simulink model "QD2_Sim_Dual"  (R2022a)
settings: Solver=FixedStepDiscrete  StartTime=0.0  StopTime=400  FixedStep=0.002  RelTol=1e-3
PreLoadFcn:
  | % QD2_Sim_Dual: agrega lib/ y sim/ al path antes de cargar (enlaces a QD2_Mission_Lib)
  | qd2_c = {pwd};
  | qd2_w = which('QD2_Sim_Dual');
  | if ~isempty(qd2_w), qd2_c{end+1} = fileparts(qd2_w); end
  | for qd2_i = 1:numel(qd2_c)
  |     qd2_d = qd2_c{qd2_i};
  |     for qd2_k = 1:4
  |         if exist(fullfile(qd2_d, 'lib', 'QD2_Mission_Lib.slx'), 'file')
  |             addpath(fullfile(qd2_d, 'lib'));
  |             addpath(fullfile(qd2_d, 'sim'));
  |             break;
  |         end
  |         qd2_d = fileparts(qd2_d);
  |     end
  | end
  | clear qd2_c qd2_w qd2_i qd2_d qd2_k
PostLoadFcn:
  | % QD2_Sim_Dual: rutas de lib/ (funciones qd2_* y QD2_Mission_Lib) y sim/
  | qd2_d = fileparts(get_param(bdroot, 'FileName'));
  | for qd2_k = 1:4
  |     if exist(fullfile(qd2_d, 'lib', 'qd2_params.m'), 'file'), break; end
  |     qd2_d = fileparts(qd2_d);
  | end
  | addpath(fullfile(qd2_d, 'lib'));
  | addpath(fullfile(qd2_d, 'sim'));
  | clear qd2_d qd2_k
InitFcn:
  | % QD2_Sim_Dual: rutas de lib/ (funciones qd2_* y QD2_Mission_Lib) y sim/
  | qd2_d = fileparts(get_param(bdroot, 'FileName'));
  | for qd2_k = 1:4
  |     if exist(fullfile(qd2_d, 'lib', 'qd2_params.m'), 'file'), break; end
  |     qd2_d = fileparts(qd2_d);
  | end
  | addpath(fullfile(qd2_d, 'lib'));
  | addpath(fullfile(qd2_d, 'sim'));
  | clear qd2_d qd2_k
  | % Parámetros (config/estacion.json es la única fuente de verdad)
  | QD2P = qd2_params_from_config();
  | QD2_SIM = qd2_sim_parametros();
  | % La versión la fija el bloque constante VERSION de la raíz
  | QD2_VERSION = str2double(get_param([bdroot '/' sprintf('VERSION\n(1 = PID, 2 = MPC)')], 'Value'));
libraries: simulink x1
(part 1 of 2)
settings Model: ExtModeTrigDuration=10000  Creator=ezequ  LastModifiedBy=ezequ
settings SolverCC: AlgebraicLoopSolver=TrustRegion  PositivePriorityOrder=on
settings DataIOCC: SaveFormat=Array  SaveOutput=off  SignalLogging=off  SaveTime=off
settings OptimizationCC: LifeSpan=inf
settings DebuggingCC: AlgebraicLoopMsg=error  UnconnectedInputMsg=warning  UnconnectedOutputMsg=warning  UnconnectedLineMsg=warning  ArithmeticOperatorsInVariantConditions=warning
settings SFSimCC: SimUseLocalCustomCode=off  CustomCodeUndefinedFunction=UseInterfaceOnly
settings RTWCC: Description=QUARC Win64 Target  SystemTargetFile=quarc_win64.tlc  TemplateMakefile=quarc_default_tmf  RTWUseLocalCustomCode=off
settings CodeAppCC: StateflowObjectComments=on
settings STFCustomTargetCC: TargetPreCompLibLocation=C:\PROGRA~3\QUARC\lib\2016a\win64\release  TargetLangStandard=C99 (ISO)  ConcurrentExecutionCompliant=on  SystemTargetFile=quarc_win64.tlc
settings GRTTargetCC: TargetPreCompLibLocation=C:\PROGRA~3\QUARC\lib\2016a\win64\release  ParMdlRefBuildCompliant=off  CompOptLevelCompliant=off  CombineOutputUpdateFcns=off  MatFileLogging=off  CPPClassGenCompliant=off  GRTInterface=on  UseToolchainInfoCompliant=off  ExtMode=on  ExtModeMexFile=quarc_comm
settings ConfigComp: CovMetricSettings=dswe  CovBoundaryAbsTol=1.0e-5

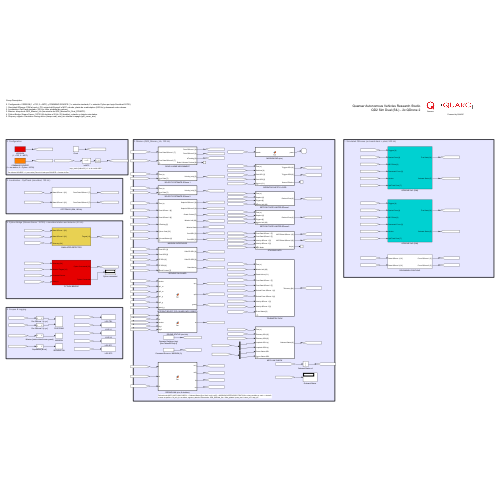
[thumbnail: Simulink's stored preview of the top-level diagram]
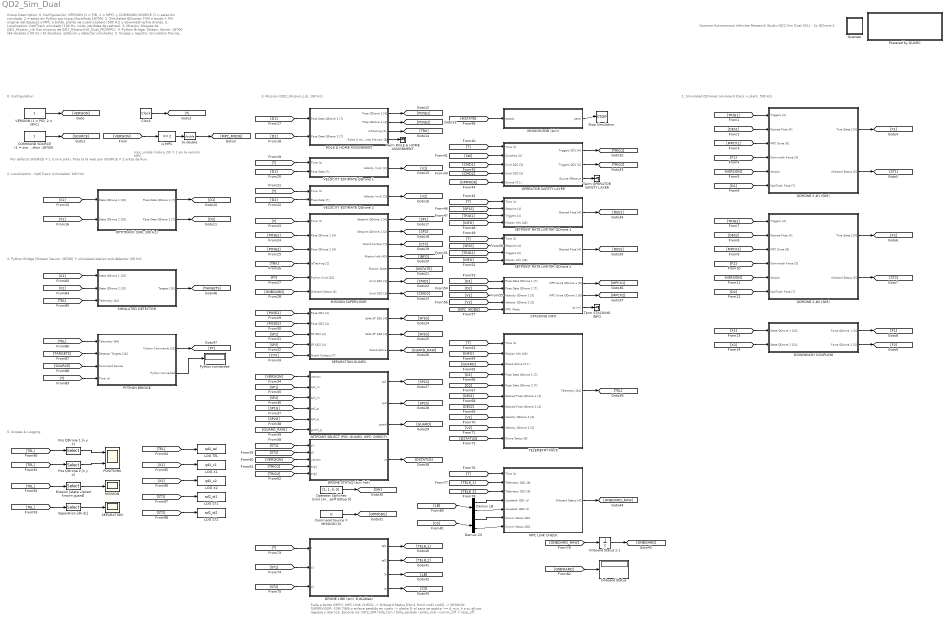
== system QD2_Sim_Dual ==
  note: Group Description:
      |
      | 0. Configuración: VERSION (1 = PID, 2 = MPC) y COMMAND SOURCE (1 = estación simulada, 2 = estación Python por tcpip://localhost:18700).
      | 1. Simulated QDrones: FSM a bordo + PIV original del Equipo2 o MPC a bordo, planta de cuadricóptero (500 Hz) y downwash entre drones.
      | 2. Localization: OptiTrack simulado (100 Hz, ruido, pérdidas de rastreo).
      | 3. Mission: bloques de QD2_Mission_Lib (los mismos de QD2_MissionCtrl_Dual_PID/MPC).
      | 4. Python Bridge: Stream Server :18700 (64 doubles a 50 Hz / 32 doubles), estación y detector simulados.
      | 5. Scopes y registro. Simulation Pacing activo (tiempo real); sim() sin interfaz lo apaga (qd2_correr_sim).
  note: Quanser Autonomous Vehicles Research Studio
      | QD2 Sim Dual (SIL) - 2x QDrone 2
  note: 0. Configuration
  note: mpc_mode (índice 23) = 1 en la versión MPC
  note: Por defecto SOURCE = 1 (corre sola). Para la UI web pon SOURCE = 2 antes de Run.
  note: 1. Simulated QDrones (on-board stack + plant, 500 Hz)
  note: 2. Localization - OptiTrack (simulated, 100 Hz)
  note: 3. Mission (QD2_Mission_Lib, 100 Hz)
  note: Falla a bordo (MPC): MPC LINK CHECK -> Onboard Status [fsm1 fsm2 cod1 cod2] -> MISSION SUPERVISOR. FSM 7/8/9 o enlace perdido en vuelo -> alerta 9:
      | el sano se aparta >= d_min_h a su altura, regresa y aterriza. Escenarios: QD2_SIM.falla_fsm / falla_apilado / proto_mal / comm_off + resp_off.
  note: 4. Python Bridge (Stream Server :18700) + simulated station and detector (50 Hz)
  note: 5. Scopes & Logging
  "COMMAND SOURCE (1 = sim station, 2 = Python :18700)" : Constant
  Clock : DigitalClock  SampleTime=0.01
  Command Source = MISSION (0) : Constant  Value=0  SampleTime=0.01
  DOWNWASH COUPLING : Subsystem
  "DRONE LINK (sim, 8 doubles)" : MATLAB Function  TreatAsAtomicUnit=on
  DRONE STATUS (sim link) : MATLAB Function  TreatAsAtomicUnit=on
  Demux CS : Demux  Outputs=2
  Demux LB : Demux  Outputs=2
  LOG ST1 : ToWorkspace  VariableName=qd2_st1  SampleTime=0.02
  LOG ST2 : ToWorkspace  VariableName=qd2_st2  SampleTime=0.02
  LOG TEL : ToWorkspace  VariableName=qd2_tel  SampleTime=0.02
  LOG X1 : ToWorkspace  VariableName=qd2_x1  SampleTime=0.02
  LOG X2 : ToWorkspace  VariableName=qd2_x2  SampleTime=0.02
  MISSION : Scope
  MISSION END (sim) : MATLAB Function  TreatAsAtomicUnit=on
  MISSION SUPERVISOR : Subsystem  TreatAsAtomicUnit=on  SystemSampleTime=Ts  mask(QD2 Mission Lib){P=QD2P, version=QD2_VERSION, Ts=0.01}
      mask prompts: P "Parámetros de misión (struct de qd2_params_from_config):"; version "Versión (1 = PID, 2 = MPC):"; Ts "Paso de muestreo (s):"
      mask help: FSM de misión (qd2_mission_step, ARQUITECTURA §3.3). Commands = [arm takeoff estop] por dron: el OPERATOR SAFETY LAYER los combina con los switches del operador. Guard Context = [explorer_id ctx_guard(6)]. Onboard Status [4] = [fsm1 fsm2 cod1 cod2] del MPC LINK CHECK (versión MPC; en PID constante 0 = desconocido; cod 1 = protocolo MPC incorrecto, 2 = enlace perdido): un dron en vuelo con FSM a bordo 7/8/9 o sin enlace (o protocolo incorrecto) -> alerta 9 (10), el sano se aparta >= d_min_h a su altura, regresa y aterriza; DONE. En LANDING, R no baja hasta que E está a >= d_min_h en horizontal. Mission Info [40] = campos de telemetría para el TELEMETRY PACK (ver codigo_supervisor en construir_modelos.m).
  MPC LINK CHECK : Subsystem  TreatAsAtomicUnit=on  SystemSampleTime=Ts  mask(QD2 Mission Lib){P=QD2P, version=QD2_VERSION, Ts=0.01}
      mask prompts: P "Parámetros de misión (struct de qd2_params_from_config):"; version "Versión (1 = PID, 2 = MPC):"; Ts "Paso de muestreo (s):"
      mask help: Versión MPC (qd2_enlace_mpc): valida la respuesta de 8 doubles de cada dron (§3.2): válida si y(8) = 2 (etiqueta protocolo MPC v1) y la FSM y(2) es un entero 1..9. Si el dron está conectado (loopback < 0.5 s y sin pérdida de enlace) y responde mal más de 0.5 s seguidos -> protocolo incorrecto (cod 1, alerta 10, dron no disponible). Sin conexión después de haber estado conectado -> enlace perdido (cod 2; la FSM retenida no se usa: fsm = 0). Onboard Status = [fsm1 fsm2 cod1 cod2] (fsm 0 = desconocida) -> MISSION SUPERVISOR. Con version = 1 (PID, el dron solo devuelve el eco) la salida es 0.
  Mission [state visited known guard] : Selector  InputPortWidth=64  IndexOptions=Index vector (dialog)  Indices=[2 10 9 11]  OutputSizes=1
  OPERATOR SAFETY LAYER : Subsystem  TreatAsAtomicUnit=on  SystemSampleTime=Ts  mask(QD2 Mission Lib){Ts=0.01}
      mask prompts: Ts "Paso de muestreo (s):"
      mask help: Versión SIMPLE (la usa QD2_Sim_Dual; interfaz de 5/3 puertos sin cambios). Los modelos de tierra usan OPERATOR SAFETY LAYER DUAL. En modo MISIÓN (Command Source = 0) arm_i = switch AND misión, takeoff_i = switch AND misión (solo tras >= 1 s armado), estop_i = switch OR misión. En modo MANUAL Equipo2 (1) el dron 1 recibe los switches (takeoff también >= 1 s después de armar) y el dron 2 solo el E-stop. El modo solo cambia con los dos drones desarmados Y los switches Arm y Takeoff abajo (nunca se dispara solo).
  "OPTITRACK (SIM, 100 Hz)" : Subsystem
  Onboard Status : Display
  Onboard Status z-1 : UnitDelay  InitialCondition=[0; 0; 0; 0]  SampleTime=0.01  HasFrameUpgradeWarning=on
  Operator Switches (sim) [Arm Takeoff EStop 0] : Constant  Value=[1; 1; 0; 0]  SampleTime=0.01
  POSITIONS : Scope  NumInputPorts=2
  PYTHON BRIDGE : Subsystem
  Pos QDrone 1 [x y z] : Selector  InputPortWidth=64  IndexOptions=Index vector (dialog)  Indices=[17 18 19]  OutputSizes=1
  Pos QDrone 2 [x y z] : Selector  InputPortWidth=64  IndexOptions=Index vector (dialog)  Indices=[35 36 37]  OutputSizes=1
  Powered by QUARC : Subsystem  mask(Powered by QUARC){}
      mask help: Double-clicking the block will open the QUARC web site.
      settings: OpenFcn=web('https://www.quanser.com/products/quarc-real-time-control-software/', '-browser');
      mask Help: web(qc_get_block_help_path(gcb));
      mask Display: image(imread(fullfile(qc_root, 'blocks', 'quarc_logo.png')));
  Python connected : Display
  QDRONE 2 #1 (SIM) : Subsystem
  QDRONE 2 #2 (SIM) : Subsystem
  Quanser : Subsystem  mask(Powered by Quanser){}
      mask help: Double-clicking the block will open the Quanser web site.
      settings: OpenFcn=web('http://www.quanser.com', '-browser');
      mask Help: web(qc_get_block_help_path(gcb));
      mask Display: image(imread(fullfile(qc_root, 'blocks', 'quanser_logo.jpg')));
  ROLE & HOME ASSIGNMENT : Subsystem  TreatAsAtomicUnit=on  SystemSampleTime=Ts  mask(QD2 Mission Lib){P=QD2P, version=QD2_VERSION, Ts=0.01}
      mask prompts: P "Parámetros de misión (struct de qd2_params_from_config):"; version "Versión (1 = PID, 2 = MPC):"; Ts "Paso de muestreo (s):"
      mask help: Separa [x y z yaw] e isTracking de cada dron (Corrected Pose Data [7] = [x y z roll pitch yaw isTracking]) y muestra en vivo la asignación de roles de qd2_assign_roles: [explorer_id responder_id home1(2) home2(2) d_homes start_ok]. El dron con menor x es el EXPLORADOR. El MISSION SUPERVISOR fija roles y homes al recibir START; start_ok = 0 avisa ANTES de START que los homes están demasiado cerca (START se rechazaría, alerta 1).
  SEPARATION : Scope
  SEPARATION GUARD : Subsystem  TreatAsAtomicUnit=on  SystemSampleTime=Ts  mask(QD2 Mission Lib){P=QD2P, Ts=0.01}
      mask prompts: P "Parámetros de misión (struct de qd2_params_from_config):"; Ts "Paso de muestreo (s):"
      mask help: Versión PID: nunca uno encima del otro (qd2_separation_guard). Distancia horizontal >= d_min_h entre poses, consignas y caminos rectos. Traduce dron <-> rol con explorer_id (Guard Context(1)) y reinicia su estado si los roles cambian. Después de este bloque la consigna DEBE limitarse por norma (SETPOINT RATE LIMITER).
  SETPOINT RATE LIMITER QDrone 1 : Subsystem  TreatAsAtomicUnit=on  SystemSampleTime=Ts  mask(QD2 Mission Lib){P=QD2P, dron=1, Ts=0.01}
      mask prompts: P "Parámetros de misión (struct de qd2_params_from_config):"; dron "QDrone (1 o 2):"; Ts "Paso de muestreo (s):"
      mask help: Saturation (como Saturation2 original, con z hasta P.z_max) + limitador de razón por NORMA en x,y (qd2_rate_limit(...,1)): 1/3 m/s xy, 1/6 m/s z, 30 °/s yaw. Sustituye al Rate Limiter2 por eje (que hace caminos en L y rompe la separación). Desarmado (Triggers(1) = 0) la consigna pasa sin limitar. Mientras este dron se aparta de un dron en falla a bordo (Mission Info(37 + dron) = 1) el límite xy es P.falla_rate_xy (1 m/s). Parámetro dron = 1 o 2.
  SETPOINT RATE LIMITER QDrone 2 : Subsystem  TreatAsAtomicUnit=on  SystemSampleTime=Ts  mask(QD2 Mission Lib){P=QD2P, dron=2, Ts=0.01}
      mask prompts: P "Parámetros de misión (struct de qd2_params_from_config):"; dron "QDrone (1 o 2):"; Ts "Paso de muestreo (s):"
      mask help: Saturation (como Saturation2 original, con z hasta P.z_max) + limitador de razón por NORMA en x,y (qd2_rate_limit(...,1)): 1/3 m/s xy, 1/6 m/s z, 30 °/s yaw. Sustituye al Rate Limiter2 por eje (que hace caminos en L y rompe la separación). Desarmado (Triggers(1) = 0) la consigna pasa sin limitar. Mientras este dron se aparta de un dron en falla a bordo (Mission Info(37 + dron) = 1) el límite xy es P.falla_rate_xy (1 m/s). Parámetro dron = 1 o 2.
  "SETPOINT SELECT (PID: GUARD, MPC: DIRECT)" : MATLAB Function  TreatAsAtomicUnit=on
  SIMULATED DETECTOR : Subsystem
  STACKING INFO : Subsystem  TreatAsAtomicUnit=on  SystemSampleTime=Ts  mask(QD2 Mission Lib){Ts=0.01}
      mask prompts: Ts "Paso de muestreo (s):"
      mask help: Versión MPC: índices 17-24 del mensaje de 24 doubles (§3.2) para cada dron = [x y z vx vy vz del OTRO dron, mpc_mode, 2]. El índice 24 = 2 es la etiqueta "protocolo MPC v1": el PROTOCOL CHECK a bordo solo acepta tramas con 24 = 2. Si el otro no está rastreado se mandan NaN (el MPC a bordo desactiva el feedforward de downwash).
  Separation [dh dz] : Selector  InputPortWidth=64  IndexOptions=Index vector (dialog)  Indices=[12 13]  OutputSizes=1
  Stop Simulation : Stop
  TELEMETRY PACK : Subsystem  TreatAsAtomicUnit=on  SystemSampleTime=Ts  mask(QD2 Mission Lib){version=QD2_VERSION, Ts=0.01}
      mask prompts: version "Versión (1 = PID, 2 = MPC):"; Ts "Paso de muestreo (s):"
      mask help: Arma los 64 doubles Simulink -> Python (§3.3) con qd2_telemetry_pack. Drone Status = [fsm1 fsm2 bat1 bat2 comm_issue1 comm_issue2 loopback1 loopback2 (n_peticiones alerta_operador)]; comm_ok = sin issue y loopback < 0.5 s. y(55) = alerta: la del operador (5-8) si hay, si no la del supervisor (0-4, 9 falla a bordo, 10 protocolo MPC incorrecto). y(56:60) = un objetivo por mensaje, rotando: [id clase x y estado]. y(61:63) = [roll pitch válido] del EXPLORADOR (rad), de Pose Data(4:5) del mismo dron (OptiTrack, R = Rz(yaw)Ry(pitch)Rx(roll)); 0 0 0 sin explorador, sin rastreo o con ángulos no finitos. y(64) = 0.
  Term OPERATOR SAFETY LAYER : Terminator
  Term ROLE & HOME ASSIGNMENT : Terminator
  Term STACKING INFO : Terminator
  VELOCITY ESTIMATE QDrone 1 : Subsystem  TreatAsAtomicUnit=on  SystemSampleTime=Ts  mask(QD2 Mission Lib){Ts=0.01}
      mask prompts: Ts "Paso de muestreo (s):"
      mask help: Velocidad [vx vy vz] a partir de OptiTrack: derivada entre muestras nuevas (100 Hz) + filtro de primer orden (tau = 0.04 s). Sin rastreo -> 0.
  VELOCITY ESTIMATE QDrone 2 : Subsystem  TreatAsAtomicUnit=on  SystemSampleTime=Ts  mask(QD2 Mission Lib){Ts=0.01}
      mask prompts: Ts "Paso de muestreo (s):"
      mask help: Velocidad [vx vy vz] a partir de OptiTrack: derivada entre muestras nuevas (100 Hz) + filtro de primer orden (tau = 0.04 s). Sin rastreo -> 0.
  "VERSION (1 = PID, 2 = MPC)" : Constant
  is MPC : simulink/Logic and Bit Operations/Compare To Constant  relop===  const=2  OutDataTypeStr=boolean
  to double : DataTypeConversion  OutDataTypeStr=double  SaturateOnIntegerOverflow=off  RndMeth=Floor
  wires:
  "VERSION (1 = PID, 2 = MPC)"/1 -> [VERSION]
  "COMMAND SOURCE (1 = sim station, 2 = Python :18700)"/1 -> [SOURCE]
  Clock/1 -> [T]
  is MPC/1 -> to double/1
  [VERSION] -> is MPC/1
  to double/1 -> [MPC_MODE]
  [TRIG1] -> QDRONE 2 #1 (SIM)/1(Triggers [4])
  [DES1] -> QDRONE 2 #1 (SIM)/2(Desired Pose [4])
  [MPCX1] -> QDRONE 2 #1 (SIM)/3(MPC Extra [8])
  [F1] -> QDRONE 2 #1 (SIM)/4(Downwash Force [3])
  [VERSION] -> QDRONE 2 #1 (SIM)/5(Version)
  [D1] -> QDRONE 2 #1 (SIM)/6(OptiTrack Pose [7])
  QDRONE 2 #1 (SIM)/1(True State [10]) -> [X1]
  QDRONE 2 #1 (SIM)/2(Onboard Status [5]) -> [ST1]
  [TRIG2] -> QDRONE 2 #2 (SIM)/1(Triggers [4])
  [DES2] -> QDRONE 2 #2 (SIM)/2(Desired Pose [4])
  [MPCX2] -> QDRONE 2 #2 (SIM)/3(MPC Extra [8])
  [F2] -> QDRONE 2 #2 (SIM)/4(Downwash Force [3])
  [VERSION] -> QDRONE 2 #2 (SIM)/5(Version)
  [D2] -> QDRONE 2 #2 (SIM)/6(OptiTrack Pose [7])
  QDRONE 2 #2 (SIM)/1(True State [10]) -> [X2]
  QDRONE 2 #2 (SIM)/2(Onboard Status [5]) -> [ST2]
  [X1] -> DOWNWASH COUPLING/1(State QDrone 1 [10])
  [X2] -> DOWNWASH COUPLING/2(State QDrone 2 [10])
  DOWNWASH COUPLING/1(Force QDrone 1 [3]) -> [F1]
  DOWNWASH COUPLING/2(Force QDrone 2 [3]) -> [F2]
  [X1] -> "OPTITRACK (SIM, 100 Hz)"/1(State QDrone 1 [10])
  [X2] -> "OPTITRACK (SIM, 100 Hz)"/2(State QDrone 2 [10])
  "OPTITRACK (SIM, 100 Hz)"/1(Pose Data QDrone 1 [7]) -> [D1]
  "OPTITRACK (SIM, 100 Hz)"/2(Pose Data QDrone 2 [7]) -> [D2]
  [D1] -> ROLE & HOME ASSIGNMENT/1(Pose Data QDrone 1 [7])
  [D2] -> ROLE & HOME ASSIGNMENT/2(Pose Data QDrone 2 [7])
  ROLE & HOME ASSIGNMENT/1(Pose QDrone 1 [4]) -> [POSE1]
  ROLE & HOME ASSIGNMENT/2(Pose QDrone 2 [4]) -> [POSE2]
  ROLE & HOME ASSIGNMENT/3(isTracking [2]) -> [TRK]
  ROLE & HOME ASSIGNMENT/4(Roles & Homes Preview [8]) -> Term ROLE & HOME ASSIGNMENT/1
  [T] -> VELOCITY ESTIMATE QDrone 1/1(Time (s))
  [D1] -> VELOCITY ESTIMATE QDrone 1/2(Pose Data [7])
  VELOCITY ESTIMATE QDrone 1/1(Velocity (m/s) [3]) -> [V1]
  [T] -> VELOCITY ESTIMATE QDrone 2/1(Time (s))
  [D2] -> VELOCITY ESTIMATE QDrone 2/2(Pose Data [7])
  VELOCITY ESTIMATE QDrone 2/1(Velocity (m/s) [3]) -> [V2]
  [T] -> MISSION SUPERVISOR/1(Time (s))
  [POSE1] -> MISSION SUPERVISOR/2(Pose QDrone 1 [4])
  [POSE2] -> MISSION SUPERVISOR/3(Pose QDrone 2 [4])
  [TRK] -> MISSION SUPERVISOR/4(isTracking [2])
  [PY] -> MISSION SUPERVISOR/5(Python Cmd [32])
  [ONBOARD] -> MISSION SUPERVISOR/6(Onboard Status [4])
  MISSION SUPERVISOR/1(Setpoint QDrone 1 [4]) -> [SP1]
  MISSION SUPERVISOR/2(Setpoint QDrone 2 [4]) -> [SP2]
  MISSION SUPERVISOR/3(Guard Context [7]) -> [CTX]
  MISSION SUPERVISOR/4(Mission Info [40]) -> [INFO]
  MISSION SUPERVISOR/5(Mission State) -> [MSTATE]
  MISSION SUPERVISOR/6(Cmd QD1 [3]) -> [CMD1]
  MISSION SUPERVISOR/7(Cmd QD2 [3]) -> [CMD2]
  [POSE1] -> SEPARATION GUARD/1(Pose QD1 [4])
  [POSE2] -> SEPARATION GUARD/2(Pose QD2 [4])
  [SP1] -> SEPARATION GUARD/3(SP QD1 [4])
  [SP2] -> SEPARATION GUARD/4(SP QD2 [4])
  [CTX] -> SEPARATION GUARD/5(Guard Context [7])
  SEPARATION GUARD/1(Safe SP QD1 [4]) -> [SP1G]
  SEPARATION GUARD/2(Safe SP QD2 [4]) -> [SP2G]
  SEPARATION GUARD/3(Guard Active) -> [GUARD_RAW]
  [VERSION] -> "SETPOINT SELECT (PID: GUARD, MPC: DIRECT)"/1(version)
  [SP1] -> "SETPOINT SELECT (PID: GUARD, MPC: DIRECT)"/2(sp1_m)
  [SP2] -> "SETPOINT SELECT (PID: GUARD, MPC: DIRECT)"/3(sp2_m)
  [SP1G] -> "SETPOINT SELECT (PID: GUARD, MPC: DIRECT)"/4(sp1_g)
  [SP2G] -> "SETPOINT SELECT (PID: GUARD, MPC: DIRECT)"/5(sp2_g)
  [GUARD_RAW] -> "SETPOINT SELECT (PID: GUARD, MPC: DIRECT)"/6(guard_g)
  "SETPOINT SELECT (PID: GUARD, MPC: DIRECT)"/1(sp1) -> [SP1S]
  "SETPOINT SELECT (PID: GUARD, MPC: DIRECT)"/2(sp2) -> [SP2S]
  "SETPOINT SELECT (PID: GUARD, MPC: DIRECT)"/3(guard) -> [GUARD]
  Operator Switches (sim) [Arm Takeoff EStop 0]/1 -> [SW]
  Command Source = MISSION (0)/1 -> [OPMODE]
  [T] -> OPERATOR SAFETY LAYER/1(Time (s))
  [SW] -> OPERATOR SAFETY LAYER/2(Switches [4])
  [CMD1] -> OPERATOR SAFETY LAYER/3(Cmd QD1 [3])
  [CMD2] -> OPERATOR SAFETY LAYER/4(Cmd QD2 [3])
  [OPMODE] -> OPERATOR SAFETY LAYER/5(Source (0,1))
  OPERATOR SAFETY LAYER/1(Triggers QD1 [4]) -> [TRIG1]
  OPERATOR SAFETY LAYER/2(Triggers QD2 [4]) -> [TRIG2]
  OPERATOR SAFETY LAYER/3(Source Effective) -> Term OPERATOR SAFETY LAYER/1
  [T] -> SETPOINT RATE LIMITER QDrone 1/1(Time (s))
  [SP1S] -> SETPOINT RATE LIMITER QDrone 1/2(Setpoint [4])
  [TRIG1] -> SETPOINT RATE LIMITER QDrone 1/3(Triggers [4])
  [INFO] -> SETPOINT RATE LIMITER QDrone 1/4(Mission Info [40])
  SETPOINT RATE LIMITER QDrone 1/1(Desired Pose [4]) -> [DES1]
  [T] -> SETPOINT RATE LIMITER QDrone 2/1(Time (s))
  [SP2S] -> SETPOINT RATE LIMITER QDrone 2/2(Setpoint [4])
  [TRIG2] -> SETPOINT RATE LIMITER QDrone 2/3(Triggers [4])
  [INFO] -> SETPOINT RATE LIMITER QDrone 2/4(Mission Info [40])
  SETPOINT RATE LIMITER QDrone 2/1(Desired Pose [4]) -> [DES2]
  [D1] -> STACKING INFO/1(Pose Data QDrone 1 [7])
  [D2] -> STACKING INFO/2(Pose Data QDrone 2 [7])
  [V1] -> STACKING INFO/3(Velocity QDrone 1 [3])
  [V2] -> STACKING INFO/4(Velocity QDrone 2 [3])
  [MPC_MODE] -> STACKING INFO/5(MPC Mode)
  STACKING INFO/1(MPC Extra QDrone 1 [8]) -> [MPCX1]
  STACKING INFO/2(MPC Extra QDrone 2 [8]) -> [MPCX2]
  STACKING INFO/3(dz (m)) -> Term STACKING INFO/1
  [ST1] -> DRONE STATUS (sim link)/1(s1)
  [ST2] -> DRONE STATUS (sim link)/2(s2)
  [VERSION] -> DRONE STATUS (sim link)/3(version)
  [TRIG1] -> DRONE STATUS (sim link)/4(trig1)
  [TRIG2] -> DRONE STATUS (sim link)/5(trig2)
  DRONE STATUS (sim link)/1(st) -> [DSTATUS]
  [T] -> TELEMETRY PACK/1(Time (s))
  [INFO] -> TELEMETRY PACK/2(Mission Info [40])
  [GUARD] -> TELEMETRY PACK/3(Guard Active (0,1))
  [D1] -> TELEMETRY PACK/4(Pose Data QDrone 1 [7])
  [D2] -> TELEMETRY PACK/5(Pose Data QDrone 2 [7])
  [DES1] -> TELEMETRY PACK/6(Desired Pose QDrone 1 [4])
  [DES2] -> TELEMETRY PACK/7(Desired Pose QDrone 2 [4])
  [V1] -> TELEMETRY PACK/8(Velocity QDrone 1 [3])
  [V2] -> TELEMETRY PACK/9(Velocity QDrone 2 [3])
  [DSTATUS] -> TELEMETRY PACK/10(Drone Status [8])
  TELEMETRY PACK/1(Telemetry [64]) -> [TEL]
  [T] -> "DRONE LINK (sim, 8 doubles)"/1(t)
  [ST1] -> "DRONE LINK (sim, 8 doubles)"/2(s1)
  [ST2] -> "DRONE LINK (sim, 8 doubles)"/3(s2)
  "DRONE LINK (sim, 8 doubles)"/1(tel1) -> [TEL8_1]
  "DRONE LINK (sim, 8 doubles)"/2(tel2) -> [TEL8_2]
  "DRONE LINK (sim, 8 doubles)"/3(lb) -> [LB]
  "DRONE LINK (sim, 8 doubles)"/4(cs) -> [CS]
  [T] -> MPC LINK CHECK/1(Time (s))
  [TEL8_1] -> MPC LINK CHECK/2(Telemetry QD1 [8])
  [TEL8_2] -> MPC LINK CHECK/3(Telemetry QD2 [8])
  MPC LINK CHECK/1(Onboard Status [4]) -> [ONBOARD_RAW]
  [ONBOARD_RAW] -> Onboard Status z-1/1
  Onboard Status z-1/1 -> [ONBOARD]
  [LB] -> Demux LB/1
  Demux LB/1 -> MPC LINK CHECK/4(Loopback QD1 (s))
  Demux LB/2 -> MPC LINK CHECK/5(Loopback QD2 (s))
  [CS] -> Demux CS/1
  Demux CS/1 -> MPC LINK CHECK/6(Comm Status QD1)
  Demux CS/2 -> MPC LINK CHECK/7(Comm Status QD2)
  [ONBOARD] -> Onboard Status/1
  [X1] -> SIMULATED DETECTOR/1(State QDrone 1 [10])
  [X2] -> SIMULATED DETECTOR/2(State QDrone 2 [10])
  [TEL] -> SIMULATED DETECTOR/3(Telemetry [64])
  SIMULATED DETECTOR/1(Targets [16]) -> [TARGETS]
  [TEL] -> PYTHON BRIDGE/1(Telemetry [64])
  [TARGETS] -> PYTHON BRIDGE/2(Detector Targets [16])
  [SOURCE] -> PYTHON BRIDGE/3(Command Source)
  [T] -> PYTHON BRIDGE/4(Time (s))
  PYTHON BRIDGE/1(Python Commands [32]) -> [PY]
  PYTHON BRIDGE/2(Python Connected) -> Python connected/1
  [TEL] -> Pos QDrone 1 [x y z]/1
  [TEL] -> Pos QDrone 2 [x y z]/1
  [TEL] -> Mission [state visited known guard]/1
  [TEL] -> Separation [dh dz]/1
  Pos QDrone 1 [x y z]/1 -> POSITIONS/1
  Pos QDrone 2 [x y z]/1 -> POSITIONS/2
  Mission [state visited known guard]/1 -> MISSION/1
  Separation [dh dz]/1 -> SEPARATION/1
  [TEL] -> LOG TEL/1
  [X1] -> LOG X1/1
  [X2] -> LOG X2/1
  [ST1] -> LOG ST1/1
  [ST2] -> LOG ST2/1
  [MSTATE] -> MISSION END (sim)/1(estado)
  MISSION END (sim)/1(parar) -> Stop Simulation/1

== system QD2_Sim_Dual/DOWNWASH COUPLING ==
  State QDrone 1 [10] : Inport
  State QDrone 2 [10] : Inport  Port=2
  Turbulence : RandomNumber  Mean=zeros(6,1)  Variance=ones(6,1)  Seed=QD2_SIM.semilla + [11 12 13 14 15 16]'  SampleTime=0.002
  qd2_downwash (both ways) : MATLAB Function  TreatAsAtomicUnit=on
  Force QDrone 1 [3] : Outport
  Force QDrone 2 [3] : Outport  Port=2
  wires:
  State QDrone 1 [10]/1 -> qd2_downwash (both ways)/1(x1)
  State QDrone 2 [10]/1 -> qd2_downwash (both ways)/2(x2)
  Turbulence/1 -> qd2_downwash (both ways)/3(n)
  qd2_downwash (both ways)/1(F1) -> Force QDrone 1 [3]/1
  qd2_downwash (both ways)/2(F2) -> Force QDrone 2 [3]/1

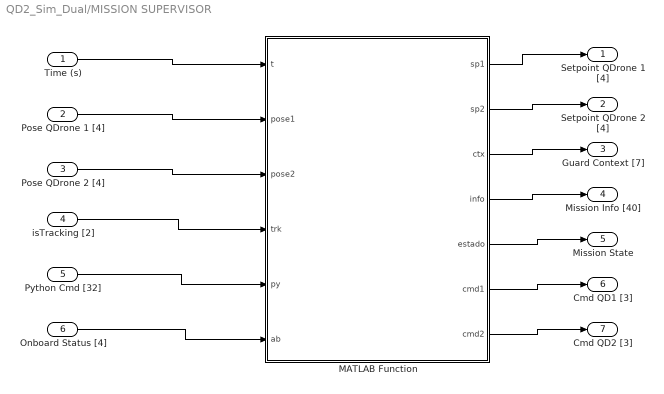
== system QD2_Sim_Dual/MISSION SUPERVISOR ==
  Time (s) : Inport
  Pose QDrone 1 [4] : Inport  Port=2
  Pose QDrone 2 [4] : Inport  Port=3
  isTracking [2] : Inport  Port=4
  Python Cmd [32] : Inport  Port=5
  Onboard Status [4] : Inport  Port=6
  MATLAB Function : MATLAB Function  TreatAsAtomicUnit=on
  Setpoint QDrone 1 [4] : Outport
  Setpoint QDrone 2 [4] : Outport  Port=2
  Guard Context [7] : Outport  Port=3
  Mission Info [40] : Outport  Port=4
  Mission State : Outport  Port=5
  Cmd QD1 [3] : Outport  Port=6
  Cmd QD2 [3] : Outport  Port=7
  wires:
  MATLAB Function/7(cmd2) -> Cmd QD2 [3]/1
  MATLAB Function/6(cmd1) -> Cmd QD1 [3]/1
  MATLAB Function/5(estado) -> Mission State/1
  MATLAB Function/4(info) -> Mission Info [40]/1
  MATLAB Function/3(ctx) -> Guard Context [7]/1
  MATLAB Function/2(sp2) -> Setpoint QDrone 2 [4]/1
  MATLAB Function/1(sp1) -> Setpoint QDrone 1 [4]/1
  Onboard Status [4]/1 -> MATLAB Function/6(ab)
  Python Cmd [32]/1 -> MATLAB Function/5(py)
  isTracking [2]/1 -> MATLAB Function/4(trk)
  Pose QDrone 2 [4]/1 -> MATLAB Function/3(pose2)
  Pose QDrone 1 [4]/1 -> MATLAB Function/2(pose1)
  Time (s)/1 -> MATLAB Function/1(t)

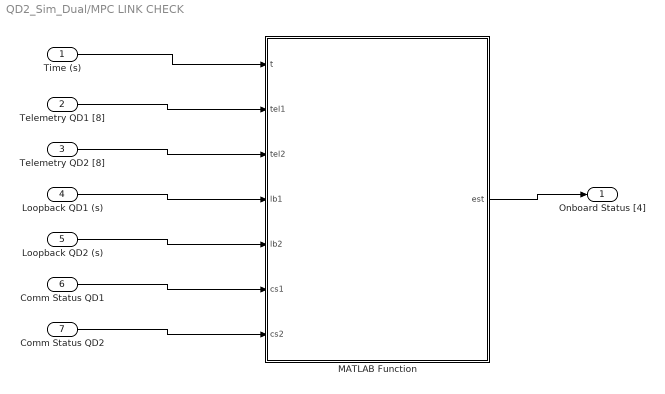
== system QD2_Sim_Dual/MPC LINK CHECK ==
  Time (s) : Inport
  Telemetry QD1 [8] : Inport  Port=2
  Telemetry QD2 [8] : Inport  Port=3
  Loopback QD1 (s) : Inport  Port=4
  Loopback QD2 (s) : Inport  Port=5
  Comm Status QD1 : Inport  Port=6
  Comm Status QD2 : Inport  Port=7
  MATLAB Function : MATLAB Function  TreatAsAtomicUnit=on
  Onboard Status [4] : Outport
  wires:
  MATLAB Function/1(est) -> Onboard Status [4]/1
  Comm Status QD2/1 -> MATLAB Function/7(cs2)
  Comm Status QD1/1 -> MATLAB Function/6(cs1)
  Loopback QD2 (s)/1 -> MATLAB Function/5(lb2)
  Loopback QD1 (s)/1 -> MATLAB Function/4(lb1)
  Telemetry QD2 [8]/1 -> MATLAB Function/3(tel2)
  Telemetry QD1 [8]/1 -> MATLAB Function/2(tel1)
  Time (s)/1 -> MATLAB Function/1(t)

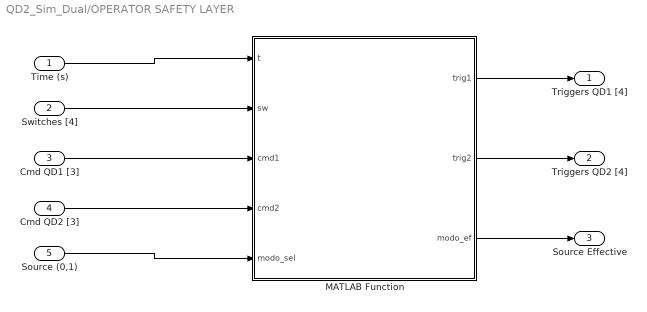
== system QD2_Sim_Dual/OPERATOR SAFETY LAYER ==
  Time (s) : Inport
  Switches [4] : Inport  Port=2
  Cmd QD1 [3] : Inport  Port=3
  Cmd QD2 [3] : Inport  Port=4
  Source (0,1) : Inport  Port=5
  MATLAB Function : MATLAB Function  TreatAsAtomicUnit=on
  Triggers QD1 [4] : Outport
  Triggers QD2 [4] : Outport  Port=2
  Source Effective : Outport  Port=3
  wires:
  MATLAB Function/3(modo_ef) -> Source Effective/1
  MATLAB Function/2(trig2) -> Triggers QD2 [4]/1
  MATLAB Function/1(trig1) -> Triggers QD1 [4]/1
  Source (0,1)/1 -> MATLAB Function/5(modo_sel)
  Cmd QD2 [3]/1 -> MATLAB Function/4(cmd2)
  Cmd QD1 [3]/1 -> MATLAB Function/3(cmd1)
  Switches [4]/1 -> MATLAB Function/2(sw)
  Time (s)/1 -> MATLAB Function/1(t)

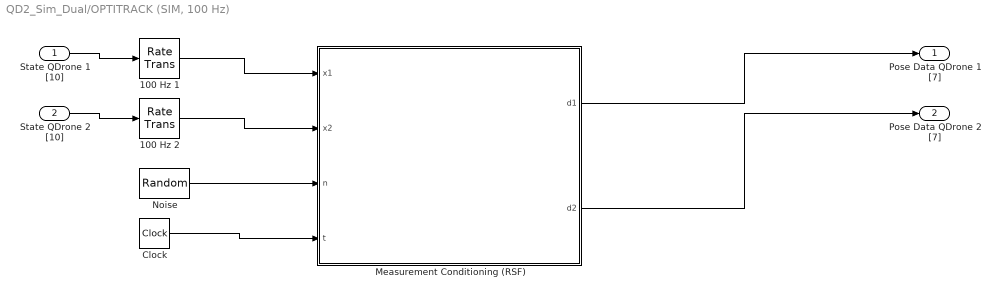
== system QD2_Sim_Dual/OPTITRACK (SIM, 100 Hz) ==
  State QDrone 1 [10] : Inport
  State QDrone 2 [10] : Inport  Port=2
  100 Hz 1 : RateTransition  OutPortSampleTime=0.01
  100 Hz 2 : RateTransition  OutPortSampleTime=0.01
  Clock : DigitalClock  SampleTime=0.01
  Measurement Conditioning (RSF) : MATLAB Function  TreatAsAtomicUnit=on
  Noise : RandomNumber  Mean=zeros(8,1)  Variance=ones(8,1)  Seed=QD2_SIM.semilla + (21:28)'  SampleTime=0.01
  Pose Data QDrone 1 [7] : Outport
  Pose Data QDrone 2 [7] : Outport  Port=2
  wires:
  State QDrone 1 [10]/1 -> 100 Hz 1/1
  State QDrone 2 [10]/1 -> 100 Hz 2/1
  100 Hz 1/1 -> Measurement Conditioning (RSF)/1(x1)
  100 Hz 2/1 -> Measurement Conditioning (RSF)/2(x2)
  Noise/1 -> Measurement Conditioning (RSF)/3(n)
  Clock/1 -> Measurement Conditioning (RSF)/4(t)
  Measurement Conditioning (RSF)/1(d1) -> Pose Data QDrone 1 [7]/1
  Measurement Conditioning (RSF)/2(d2) -> Pose Data QDrone 2 [7]/1

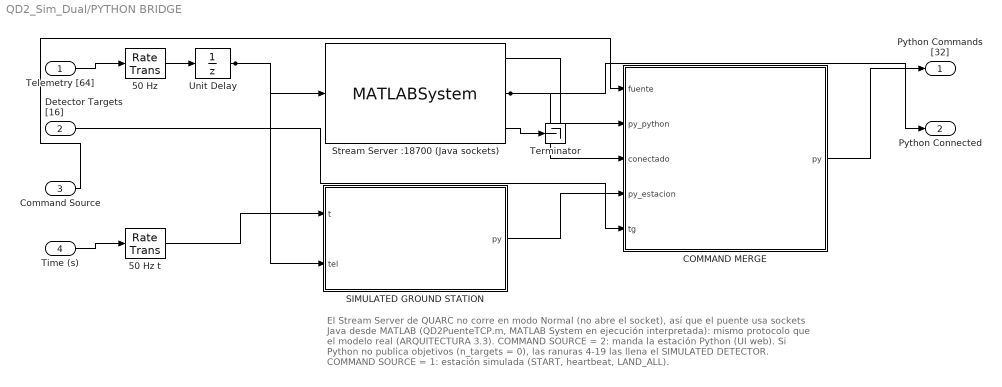
== system QD2_Sim_Dual/PYTHON BRIDGE ==
  note: El Stream Server de QUARC no corre en modo Normal (no abre el socket), así que el puente usa sockets Java desde MATLAB
      | (QD2PuenteTCP.m, MATLAB System en ejecución interpretada): mismo protocolo que el modelo real (ARQUITECTURA 3.3).
      | COMMAND SOURCE = 2: manda la estación Python (UI web). Si Python no publica objetivos (n_targets = 0), las
      | ranuras 4-19 las llena el SIMULATED DETECTOR. COMMAND SOURCE = 1: estación simulada (START, heartbeat, LAND_ALL).
  Telemetry [64] : Inport
  Detector Targets [16] : Inport  Port=2
  Command Source : Inport  Port=3
  Time (s) : Inport  Port=4
  50 Hz : RateTransition  OutPortSampleTime=0.02
  50 Hz t : RateTransition  OutPortSampleTime=0.02
  COMMAND MERGE : MATLAB Function  TreatAsAtomicUnit=on
  SIMULATED GROUND STATION : MATLAB Function  TreatAsAtomicUnit=on
  Stream Server :18700 (Java sockets) : MATLABSystem  System=QD2PuenteTCP  Puerto=QD2_SIM.puerto  Direccion=127.0.0.1  Activo=1  TDesconectar=5  Ts=0.02
      mask Type: QD2PuenteTCP
      mask Display:
      | disp('QD2PuenteTCP');
      | port_label('input',1,'Telemetry [64]');
      | port_label('output',1,'Python Commands [32]');
      | port_label('output',2,'Connected');
      | port_label('output',3,'Packets Rx');
  Terminator : Terminator
  Unit Delay : UnitDelay  InitialCondition=zeros(64,1)  SampleTime=0.02  HasFrameUpgradeWarning=on
  Python Commands [32] : Outport
  Python Connected : Outport  Port=2
  wires:
  Telemetry [64]/1 -> 50 Hz/1
  50 Hz/1 -> Unit Delay/1
  Unit Delay/1 -> Stream Server :18700 (Java sockets)/1, SIMULATED GROUND STATION/2(tel)
  Time (s)/1 -> 50 Hz t/1
  50 Hz t/1 -> SIMULATED GROUND STATION/1(t)
  Command Source/1 -> COMMAND MERGE/1(fuente)
  Stream Server :18700 (Java sockets)/1 -> COMMAND MERGE/2(py_python)
  Stream Server :18700 (Java sockets)/2 -> COMMAND MERGE/3(conectado), Python Connected/1
  SIMULATED GROUND STATION/1(py) -> COMMAND MERGE/4(py_estacion)
  Detector Targets [16]/1 -> COMMAND MERGE/5(tg)
  COMMAND MERGE/1(py) -> Python Commands [32]/1
  Stream Server :18700 (Java sockets)/3 -> Terminator/1

== system QD2_Sim_Dual/Powered by QUARC ==
  EmptySubsystem : Subsystem

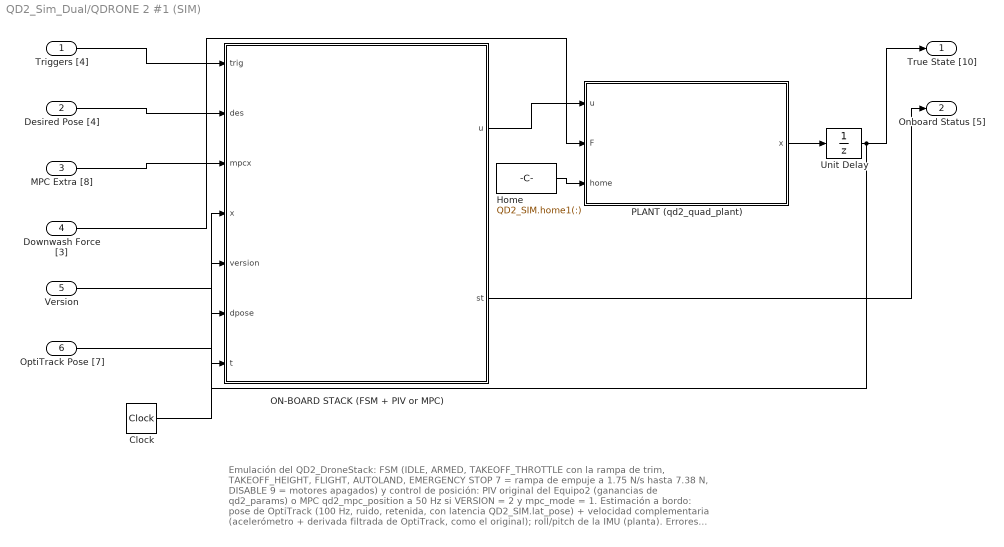
== system QD2_Sim_Dual/QDRONE 2 #1 (SIM) ==
  note: Emulación del QD2_DroneStack: FSM (IDLE, ARMED, TAKEOFF_THROTTLE con la rampa de trim, TAKEOFF_HEIGHT, FLIGHT, AUTOLAND,
      | EMERGENCY STOP 7 = rampa de empuje a 1.75 N/s hasta 7.38 N, DISABLE 9 = motores apagados) y control de posición: PIV original del
      | Equipo2 (ganancias de qd2_params) o MPC qd2_mpc_position a 50 Hz si VERSION = 2 y mpc_mode = 1.
      | Estimación a bordo: pose de OptiTrack (100 Hz, ruido, retenida, con latencia QD2_SIM.lat_pose) + velocidad complementaria
      | (acelerómetro + derivada filtrada de OptiTrack, como el original); roll/pitch de la IMU (planta). Errores como el original:
      | isTracking = 0 durante 0.2 s -> 7; enlace caído (QD2_SIM.comm_off) 0.5 s -> 7 y 1 s armado -> 9 (FLIGHT SAFETY corta motores).
      | Fallas a bordo programadas: QD2_SIM.falla_fsm [dron t] o QD2_SIM.falla_apilado (1 = el de arriba, 2 = el de abajo) -> 7.
      | Onboard Status = [FSM, batería (V), estado MPC (0 ok, 3 inactivo, 4 PIV), empuje (N), comm issue].
      | True State = [x y z vx vy vz roll pitch yaw T]. El STABILIZER se aproxima con la actitud de 1er orden de la planta.
  Triggers [4] : Inport
  Desired Pose [4] : Inport  Port=2
  MPC Extra [8] : Inport  Port=3
  Downwash Force [3] : Inport  Port=4
  Version : Inport  Port=5
  OptiTrack Pose [7] : Inport  Port=6
  Clock : DigitalClock  SampleTime=0.002
  Home : Constant  Value=QD2_SIM.home1(:)
  ON-BOARD STACK (FSM + PIV or MPC) : MATLAB Function  TreatAsAtomicUnit=on
  PLANT (qd2_quad_plant) : MATLAB Function  TreatAsAtomicUnit=on
  Unit Delay : UnitDelay  InitialCondition=[QD2_SIM.home1(:); zeros(8,1)]  SampleTime=0.002  HasFrameUpgradeWarning=on
  True State [10] : Outport
  Onboard Status [5] : Outport  Port=2
  wires:
  Triggers [4]/1 -> ON-BOARD STACK (FSM + PIV or MPC)/1(trig)
  Desired Pose [4]/1 -> ON-BOARD STACK (FSM + PIV or MPC)/2(des)
  MPC Extra [8]/1 -> ON-BOARD STACK (FSM + PIV or MPC)/3(mpcx)
  Unit Delay/1 -> ON-BOARD STACK (FSM + PIV or MPC)/4(x), True State [10]/1
  Version/1 -> ON-BOARD STACK (FSM + PIV or MPC)/5(version)
  OptiTrack Pose [7]/1 -> ON-BOARD STACK (FSM + PIV or MPC)/6(dpose)
  Clock/1 -> ON-BOARD STACK (FSM + PIV or MPC)/7(t)
  ON-BOARD STACK (FSM + PIV or MPC)/1(u) -> PLANT (qd2_quad_plant)/1(u)
  Downwash Force [3]/1 -> PLANT (qd2_quad_plant)/2(F)
  Home/1 -> PLANT (qd2_quad_plant)/3(home)
  PLANT (qd2_quad_plant)/1(x) -> Unit Delay/1
  ON-BOARD STACK (FSM + PIV or MPC)/2(st) -> Onboard Status [5]/1

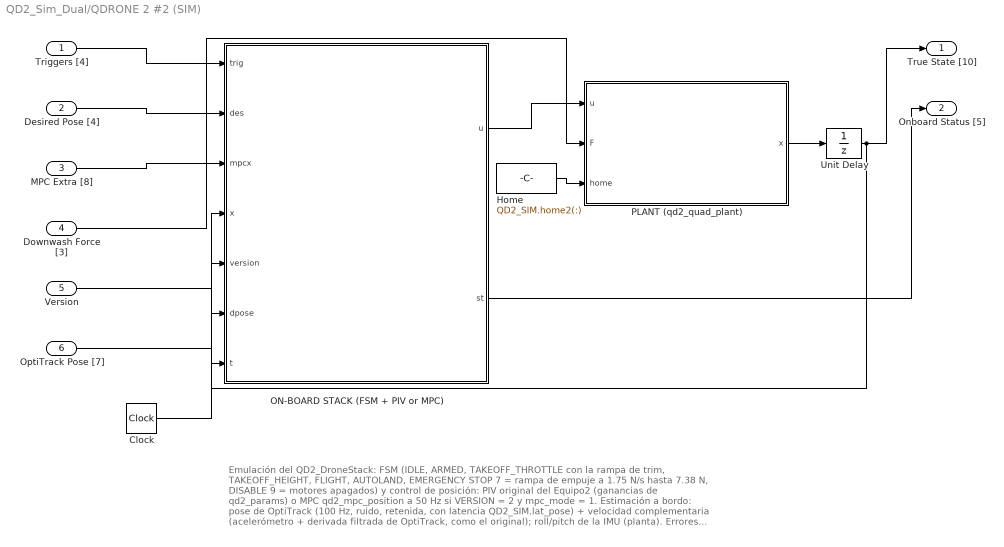
== system QD2_Sim_Dual/QDRONE 2 #2 (SIM) ==
  note: Emulación del QD2_DroneStack: FSM (IDLE, ARMED, TAKEOFF_THROTTLE con la rampa de trim, TAKEOFF_HEIGHT, FLIGHT, AUTOLAND,
      | EMERGENCY STOP 7 = rampa de empuje a 1.75 N/s hasta 7.38 N, DISABLE 9 = motores apagados) y control de posición: PIV original del
      | Equipo2 (ganancias de qd2_params) o MPC qd2_mpc_position a 50 Hz si VERSION = 2 y mpc_mode = 1.
      | Estimación a bordo: pose de OptiTrack (100 Hz, ruido, retenida, con latencia QD2_SIM.lat_pose) + velocidad complementaria
      | (acelerómetro + derivada filtrada de OptiTrack, como el original); roll/pitch de la IMU (planta). Errores como el original:
      | isTracking = 0 durante 0.2 s -> 7; enlace caído (QD2_SIM.comm_off) 0.5 s -> 7 y 1 s armado -> 9 (FLIGHT SAFETY corta motores).
      | Fallas a bordo programadas: QD2_SIM.falla_fsm [dron t] o QD2_SIM.falla_apilado (1 = el de arriba, 2 = el de abajo) -> 7.
      | Onboard Status = [FSM, batería (V), estado MPC (0 ok, 3 inactivo, 4 PIV), empuje (N), comm issue].
      | True State = [x y z vx vy vz roll pitch yaw T]. El STABILIZER se aproxima con la actitud de 1er orden de la planta.
  Triggers [4] : Inport
  Desired Pose [4] : Inport  Port=2
  MPC Extra [8] : Inport  Port=3
  Downwash Force [3] : Inport  Port=4
  Version : Inport  Port=5
  OptiTrack Pose [7] : Inport  Port=6
  Clock : DigitalClock  SampleTime=0.002
  Home : Constant  Value=QD2_SIM.home2(:)
  ON-BOARD STACK (FSM + PIV or MPC) : MATLAB Function  TreatAsAtomicUnit=on
  PLANT (qd2_quad_plant) : MATLAB Function  TreatAsAtomicUnit=on
  Unit Delay : UnitDelay  InitialCondition=[QD2_SIM.home2(:); zeros(8,1)]  SampleTime=0.002  HasFrameUpgradeWarning=on
  True State [10] : Outport
  Onboard Status [5] : Outport  Port=2
  wires:
  Triggers [4]/1 -> ON-BOARD STACK (FSM + PIV or MPC)/1(trig)
  Desired Pose [4]/1 -> ON-BOARD STACK (FSM + PIV or MPC)/2(des)
  MPC Extra [8]/1 -> ON-BOARD STACK (FSM + PIV or MPC)/3(mpcx)
  Unit Delay/1 -> ON-BOARD STACK (FSM + PIV or MPC)/4(x), True State [10]/1
  Version/1 -> ON-BOARD STACK (FSM + PIV or MPC)/5(version)
  OptiTrack Pose [7]/1 -> ON-BOARD STACK (FSM + PIV or MPC)/6(dpose)
  Clock/1 -> ON-BOARD STACK (FSM + PIV or MPC)/7(t)
  ON-BOARD STACK (FSM + PIV or MPC)/1(u) -> PLANT (qd2_quad_plant)/1(u)
  Downwash Force [3]/1 -> PLANT (qd2_quad_plant)/2(F)
  Home/1 -> PLANT (qd2_quad_plant)/3(home)
  PLANT (qd2_quad_plant)/1(x) -> Unit Delay/1
  ON-BOARD STACK (FSM + PIV or MPC)/2(st) -> Onboard Status [5]/1

== system QD2_Sim_Dual/Quanser ==
  EmptySubsystem : Subsystem

== system QD2_Sim_Dual/ROLE & HOME ASSIGNMENT ==
  Pose Data QDrone 1 [7] : Inport
  Pose Data QDrone 2 [7] : Inport  Port=2
  MATLAB Function : MATLAB Function  TreatAsAtomicUnit=on
  Pose QDrone 1 [4] : Outport
  Pose QDrone 2 [4] : Outport  Port=2
  isTracking [2] : Outport  Port=3
  Roles & Homes Preview [8] : Outport  Port=4
  wires:
  MATLAB Function/4(prev) -> Roles & Homes Preview [8]/1
  MATLAB Function/3(trk) -> isTracking [2]/1
  MATLAB Function/2(pose2) -> Pose QDrone 2 [4]/1
  MATLAB Function/1(pose1) -> Pose QDrone 1 [4]/1
  Pose Data QDrone 2 [7]/1 -> MATLAB Function/2(d2)
  Pose Data QDrone 1 [7]/1 -> MATLAB Function/1(d1)

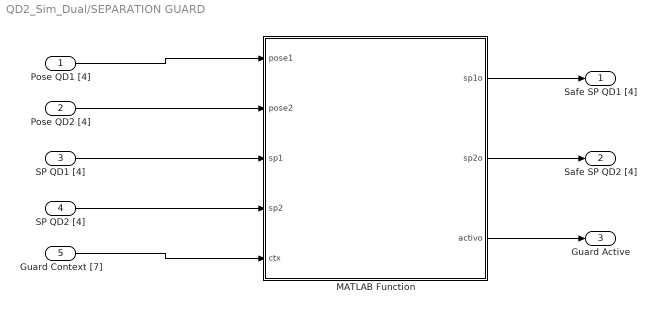
== system QD2_Sim_Dual/SEPARATION GUARD ==
  Pose QD1 [4] : Inport
  Pose QD2 [4] : Inport  Port=2
  SP QD1 [4] : Inport  Port=3
  SP QD2 [4] : Inport  Port=4
  Guard Context [7] : Inport  Port=5
  MATLAB Function : MATLAB Function  TreatAsAtomicUnit=on
  Safe SP QD1 [4] : Outport
  Safe SP QD2 [4] : Outport  Port=2
  Guard Active : Outport  Port=3
  wires:
  MATLAB Function/3(activo) -> Guard Active/1
  MATLAB Function/2(sp2o) -> Safe SP QD2 [4]/1
  MATLAB Function/1(sp1o) -> Safe SP QD1 [4]/1
  Guard Context [7]/1 -> MATLAB Function/5(ctx)
  SP QD2 [4]/1 -> MATLAB Function/4(sp2)
  SP QD1 [4]/1 -> MATLAB Function/3(sp1)
  Pose QD2 [4]/1 -> MATLAB Function/2(pose2)
  Pose QD1 [4]/1 -> MATLAB Function/1(pose1)

== system QD2_Sim_Dual/SETPOINT RATE LIMITER QDrone 1 ==
  Time (s) : Inport
  Setpoint [4] : Inport  Port=2
  Triggers [4] : Inport  Port=3
  Mission Info [40] : Inport  Port=4
  MATLAB Function : MATLAB Function  TreatAsAtomicUnit=on
  Saturation : Saturate  UpperLimit=[P.xy_lim(2); P.xy_lim(2); P.z_max; 3*pi]  LowerLimit=[P.xy_lim(1); P.xy_lim(1); 0; -3*pi]
  Desired Pose [4] : Outport
  wires:
  MATLAB Function/1(y) -> Desired Pose [4]/1
  Mission Info [40]/1 -> MATLAB Function/4(info)
  Triggers [4]/1 -> MATLAB Function/3(trig)
  Saturation/1 -> MATLAB Function/2(u)
  Setpoint [4]/1 -> Saturation/1
  Time (s)/1 -> MATLAB Function/1(t)

== system QD2_Sim_Dual/SETPOINT RATE LIMITER QDrone 2 ==
  Time (s) : Inport
  Setpoint [4] : Inport  Port=2
  Triggers [4] : Inport  Port=3
  Mission Info [40] : Inport  Port=4
  MATLAB Function : MATLAB Function  TreatAsAtomicUnit=on
  Saturation : Saturate  UpperLimit=[P.xy_lim(2); P.xy_lim(2); P.z_max; 3*pi]  LowerLimit=[P.xy_lim(1); P.xy_lim(1); 0; -3*pi]
  Desired Pose [4] : Outport
  wires:
  MATLAB Function/1(y) -> Desired Pose [4]/1
  Mission Info [40]/1 -> MATLAB Function/4(info)
  Triggers [4]/1 -> MATLAB Function/3(trig)
  Saturation/1 -> MATLAB Function/2(u)
  Setpoint [4]/1 -> Saturation/1
  Time (s)/1 -> MATLAB Function/1(t)

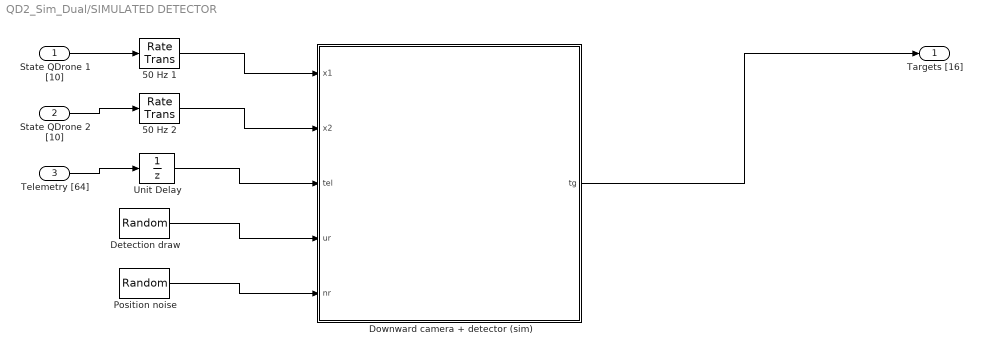
== system QD2_Sim_Dual/SIMULATED DETECTOR ==
  State QDrone 1 [10] : Inport
  State QDrone 2 [10] : Inport  Port=2
  Telemetry [64] : Inport  Port=3
  50 Hz 1 : RateTransition  OutPortSampleTime=0.02
  50 Hz 2 : RateTransition  OutPortSampleTime=0.02
  Detection draw : UniformRandomNumber  Minimum=zeros(16,1)  Maximum=ones(16,1)  Seed=QD2_SIM.semilla + (31:46)'  SampleTime=0.02
  Downward camera + detector (sim) : MATLAB Function  TreatAsAtomicUnit=on
  Position noise : RandomNumber  Mean=zeros(2,1)  Variance=ones(2,1)  Seed=QD2_SIM.semilla + [51; 52]  SampleTime=0.02
  Unit Delay : UnitDelay  InitialCondition=zeros(64,1)  SampleTime=0.02  HasFrameUpgradeWarning=on
  Targets [16] : Outport
  wires:
  State QDrone 1 [10]/1 -> 50 Hz 1/1
  State QDrone 2 [10]/1 -> 50 Hz 2/1
  Telemetry [64]/1 -> Unit Delay/1
  50 Hz 1/1 -> Downward camera + detector (sim)/1(x1)
  50 Hz 2/1 -> Downward camera + detector (sim)/2(x2)
  Unit Delay/1 -> Downward camera + detector (sim)/3(tel)
  Detection draw/1 -> Downward camera + detector (sim)/4(ur)
  Position noise/1 -> Downward camera + detector (sim)/5(nr)
  Downward camera + detector (sim)/1(tg) -> Targets [16]/1

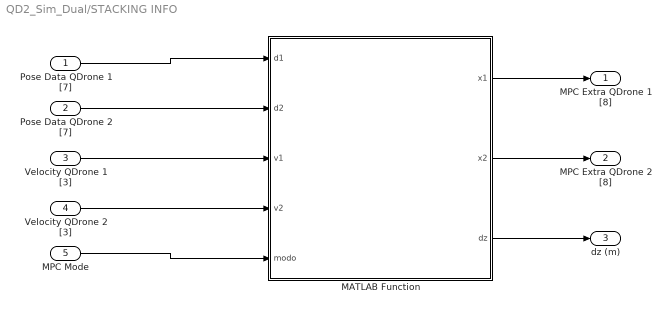
== system QD2_Sim_Dual/STACKING INFO ==
  Pose Data QDrone 1 [7] : Inport
  Pose Data QDrone 2 [7] : Inport  Port=2
  Velocity QDrone 1 [3] : Inport  Port=3
  Velocity QDrone 2 [3] : Inport  Port=4
  MPC Mode : Inport  Port=5
  MATLAB Function : MATLAB Function  TreatAsAtomicUnit=on
  MPC Extra QDrone 1 [8] : Outport
  MPC Extra QDrone 2 [8] : Outport  Port=2
  dz (m) : Outport  Port=3
  wires:
  MATLAB Function/3(dz) -> dz (m)/1
  MATLAB Function/2(x2) -> MPC Extra QDrone 2 [8]/1
  MATLAB Function/1(x1) -> MPC Extra QDrone 1 [8]/1
  MPC Mode/1 -> MATLAB Function/5(modo)
  Velocity QDrone 2 [3]/1 -> MATLAB Function/4(v2)
  Velocity QDrone 1 [3]/1 -> MATLAB Function/3(v1)
  Pose Data QDrone 2 [7]/1 -> MATLAB Function/2(d2)
  Pose Data QDrone 1 [7]/1 -> MATLAB Function/1(d1)

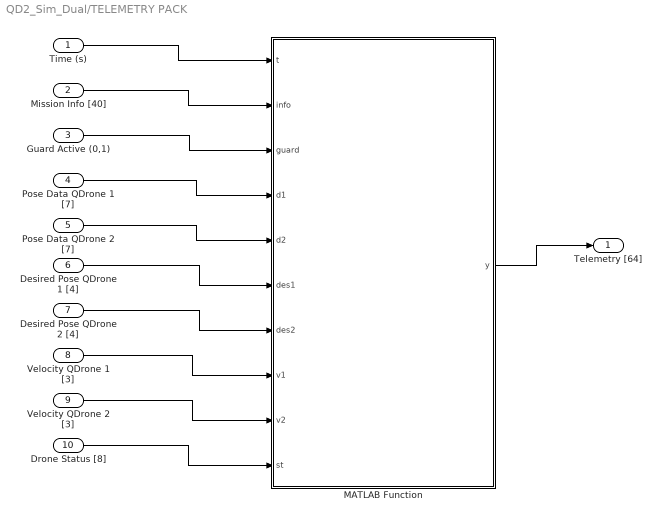
== system QD2_Sim_Dual/TELEMETRY PACK ==
  Time (s) : Inport
  Mission Info [40] : Inport  Port=2
  Guard Active (0,1) : Inport  Port=3
  Pose Data QDrone 1 [7] : Inport  Port=4
  Pose Data QDrone 2 [7] : Inport  Port=5
  Desired Pose QDrone 1 [4] : Inport  Port=6
  Desired Pose QDrone 2 [4] : Inport  Port=7
  Velocity QDrone 1 [3] : Inport  Port=8
  Velocity QDrone 2 [3] : Inport  Port=9
  Drone Status [8] : Inport  Port=10
  MATLAB Function : MATLAB Function  TreatAsAtomicUnit=on
  Telemetry [64] : Outport
  wires:
  MATLAB Function/1(y) -> Telemetry [64]/1
  Drone Status [8]/1 -> MATLAB Function/10(st)
  Velocity QDrone 2 [3]/1 -> MATLAB Function/9(v2)
  Velocity QDrone 1 [3]/1 -> MATLAB Function/8(v1)
  Desired Pose QDrone 2 [4]/1 -> MATLAB Function/7(des2)
  Desired Pose QDrone 1 [4]/1 -> MATLAB Function/6(des1)
  Pose Data QDrone 2 [7]/1 -> MATLAB Function/5(d2)
  Pose Data QDrone 1 [7]/1 -> MATLAB Function/4(d1)
  Guard Active (0,1)/1 -> MATLAB Function/3(guard)
  Mission Info [40]/1 -> MATLAB Function/2(info)
  Time (s)/1 -> MATLAB Function/1(t)

== system QD2_Sim_Dual/VELOCITY ESTIMATE QDrone 1 ==
  Time (s) : Inport
  Pose Data [7] : Inport  Port=2
  MATLAB Function : MATLAB Function  TreatAsAtomicUnit=on
  Velocity (m/s) [3] : Outport
  wires:
  MATLAB Function/1(v) -> Velocity (m/s) [3]/1
  Pose Data [7]/1 -> MATLAB Function/2(d)
  Time (s)/1 -> MATLAB Function/1(t)

== system QD2_Sim_Dual/VELOCITY ESTIMATE QDrone 2 ==
  Time (s) : Inport
  Pose Data [7] : Inport  Port=2
  MATLAB Function : MATLAB Function  TreatAsAtomicUnit=on
  Velocity (m/s) [3] : Outport
  wires:
  MATLAB Function/1(v) -> Velocity (m/s) [3]/1
  Pose Data [7]/1 -> MATLAB Function/2(d)
  Time (s)/1 -> MATLAB Function/1(t)

== system QD2_Sim_Dual/Powered by QUARC/EmptySubsystem ==

== system QD2_Sim_Dual/Quanser/EmptySubsystem ==

== matlab function QD2_Sim_Dual/DRONE STATUS (sim link) ==
  data: s1 input; st output size=[8 1]; s2 input; version input; trig1 input; trig2 input
function st = fcn(s1, s2, version, trig1, trig2)
%#codegen
% Drone Status [8] para el TELEMETRY PACK: [fsm1 fsm2 bat1 bat2 comm_issue1
% comm_issue2 loopback1 loopback2]. comm_issue viene de la emulación a bordo
% (pérdidas programadas QD2_SIM.comm_off); loopback = 0 (sin latencia de red).
% fsm (o+2 de la telemetría, ARQUITECTURA §3.3) según la versión, como los
% modelos de tierra: PID = Flight State de TIERRA (Flight Plan del Equipo2:
% 0 Idle, 1 Armed, 2 Takeoff, 3 Land, 9 MS Stop) con los disparos efectivos
% trig = [arm takeoff estop 0] y comm_issue; MPC = FSM a bordo (1..9).
persistent fp
if isempty(fp)
    fp = [0; 0];
end
fp(1) = flight_plan(fp(1), trig1, s1(5));
fp(2) = flight_plan(fp(2), trig2, s2(5));
if version < 1.5
    f1 = fp(1); f2 = fp(2);
else
    f1 = s1(1); f2 = s2(1);
end
st = [f1; f2; s1(2); s2(2); s1(5); s2(5); 0; 0];
end

function e = flight_plan(e, trig, com)
% Copia de Flight_Plan (QD2_MissionCtrl_NoJoystick_2021a/Subsystem), joystick_issue = 0.
arm = trig(1) > 0.5; tk = trig(2) > 0.5; es = trig(3) > 0.5; ci = com > 0.5;
if e == 0
    if arm && ~es
        e = 1;
    elseif es || tk || ci
        e = 9;
    end
elseif e == 1
    if ~es
        if ~arm
            e = 0;
        elseif tk
            e = 2;
        end
    elseif ci || es
        e = 9;
    end
elseif e == 2
    if ~es
        if ~tk
            e = 3;
        elseif ~arm || ci
            e = 9;
        end
    end
elseif e == 3
    if ~arm || ci
        e = 9;
    end
end
end

== matlab function QD2_Sim_Dual/DRONE LINK (sim, 8 doubles) ==
  data: t input; tel1 output size=[8 1]; s1 input; s2 input; tel2 output size=[8 1]; lb output size=[2 1]; cs output size=[2 1]; QD2_SIM parameter
function [tel1, tel2, lb, cs] = fcn(t, s1, s2, QD2_SIM)
%#codegen
% DRONE LINK (sim): respuesta de 8 doubles de cada dron como la manda
% QD2_DroneStack_MPC (ARQUITECTURA §3.2): [eco ts, FSM, batería, estado MPC, T,
% roll, pitch, 2 = etiqueta protocolo MPC v1]. s1/s2 = Onboard Status [FSM bat est T comm].
% QD2_SIM.proto_mal [dron t1 t2]: ese dron responde sin la etiqueta (0) en [t1, t2).
% QD2_SIM.resp_off [dron t1 t2]: la respuesta dron->PC no llega en [t1, t2): el Stream
% Server ("most recent") retiene la última y el loopback crece (lb = t - eco retenido).
% lb = loopback (0: el enlace simulado no tiene latencia); cs = Communication Status
% (1 si el dron perdió el enlace PC->dron, QD2_SIM.comm_off).
persistent u1 u2
if isempty(u1)
    u1 = [0; NaN(7, 1)];
    u2 = [0; NaN(7, 1)];
end
tg = [2 2];
pm = QD2_SIM.proto_mal;
for k = 1:size(pm, 1)
    if pm(k,1) >= 1 && pm(k,1) <= 2 && t >= pm(k,2) && t < pm(k,3)
        tg(pm(k,1)) = 0;
    end
end
perd = [false false];
ro = QD2_SIM.resp_off;
for k = 1:size(ro, 1)
    if ro(k,1) >= 1 && ro(k,1) <= 2 && t >= ro(k,2) && t < ro(k,3)
        perd(ro(k,1)) = true;
    end
end
lb = [0; 0];
if ~perd(1)
    u1 = [t; s1(1); s1(2); s1(3); s1(4); 0; 0; tg(1)];
else
    lb(1) = t - u1(1);
end
if ~perd(2)
    u2 = [t; s2(1); s2(2); s2(3); s2(4); 0; 0; tg(2)];
else
    lb(2) = t - u2(1);
end
tel1 = u1;
tel2 = u2;
cs = [s1(5); s2(5)];

== matlab function QD2_Sim_Dual/SIMULATED DETECTOR/Downward camera + detector (sim) ==
  data: x1 input; tg output size=[16 1]; x2 input; tel input; ur input; nr input; QD2_SIM parameter
function tg = fcn(x1, x2, tel, ur, nr, QD2_SIM)
%#codegen
% DETECTOR SIMULADO: cámara cenital del EXPLORADOR (RealSense mirando abajo).
% Huella = rectángulo de semiancho z*tan(vfov/2) (eje x del dron) por
% z*tan(hfov/2) (eje y), centrado en la cámara (offset del soporte).
% Cada objetivo dentro de la huella cuenta una observación por frame
% (~12.5 fps) con probabilidad det_p; con det_frames observaciones se
% publica como lo haría la estación Python: [id clase x y confianza].
% Salida tg = [n_targets; 3 ranuras x 5] (índices 4-19 del paquete de 32),
% rotando las ranuras entre todos los publicados.
persistent obs pub npub k rot
if isempty(obs)
    obs = zeros(16, 1);
    pub = zeros(16, 5);
    npub = 0;
    k = 0;
    rot = 0;
end
k = k + 1;
O = QD2_SIM.objetivos_tabla;
eid = tel(4);
estado = tel(2);
if mod(k, 4) == 0 && (eid == 1 || eid == 2) && estado >= 4 && estado <= 6
    if eid == 1
        xe = x1;
    else
        xe = x2;
    end
    z = xe(3);
    if z >= QD2_SIM.det_z_min
        c = cos(xe(9)); s = sin(xe(9));
        cx = xe(1) + c*QD2_SIM.det_offset(1) - s*QD2_SIM.det_offset(2);
        cy = xe(2) + s*QD2_SIM.det_offset(1) + c*QD2_SIM.det_offset(2);
        hx = z*tan(QD2_SIM.det_vfov*pi/360);
        hy = z*tan(QD2_SIM.det_hfov*pi/360);
        for j = 1:16
            if isfinite(O(j,1)) && obs(j) < QD2_SIM.det_frames
                dx = O(j,1) - cx; dy = O(j,2) - cy;
                bx = c*dx + s*dy; by = -s*dx + c*dy;
                if abs(bx) <= hx && abs(by) <= hy && ur(j) < QD2_SIM.det_p
                    obs(j) = obs(j) + 1;
                    if obs(j) >= QD2_SIM.det_frames && npub < 16
                        npub = npub + 1;
                        pub(npub, :) = [npub, O(j,3), O(j,1) + QD2_SIM.det_ruido*nr(1), ...
                                        O(j,2) + QD2_SIM.det_ruido*nr(2), 0.85];
                    end
                end
            end
        end
    end
end
tg = zeros(16, 1);
tg(1) = npub;
if npub > 0
    rot = rot + 1;
    for r = 1:3
        q = mod(rot*3 + r - 1, npub) + 1;
        tg(2 + 5*(r-1) : 6 + 5*(r-1)) = pub(q, :)';
    end
end

== matlab function QD2_Sim_Dual/PYTHON BRIDGE/SIMULATED GROUND STATION ==
  data: t input; py output size=[32 1]; tel input; QD2P parameter; QD2_SIM parameter
function py = fcn(t, tel, QD2P, QD2_SIM)
%#codegen
% ESTACIÓN SIMULADA (para correr sin la UI): heartbeat a 50 Hz, START en
% QD2_SIM.t_start y LAND_ALL cuando los dos drones llevan t_land_espera s en
% su home durante RETURN_HOME (si auto_land = false).
persistent hb seq cmd t_casa start_ok land_ok
if isempty(hb)
    hb = 0; seq = 0; cmd = 0; t_casa = -1; start_ok = 0; land_ok = 0;
end
hb = hb + 1;
estado = tel(2);
if start_ok < 0.5 && t >= QD2_SIM.t_start && estado == 2
    seq = seq + 1; cmd = 1; start_ok = 1;
end
en_casa = false;
if estado == 6
    d1 = hypot(tel(17) - tel(29), tel(18) - tel(30));
    d2 = hypot(tel(35) - tel(47), tel(36) - tel(48));
    en_casa = d1 < 0.15 && d2 < 0.15;
end
if en_casa
    if t_casa < 0, t_casa = t; end
else
    t_casa = -1;
end
if land_ok < 0.5 && QD2P.auto_land < 0.5 && t_casa >= 0 && t - t_casa >= QD2_SIM.t_land_espera
    seq = seq + 1; cmd = 3; land_ok = 1;
end
py = zeros(32, 1);
py(1) = hb;
py(2) = cmd;
py(3) = seq;

== matlab function QD2_Sim_Dual/PYTHON BRIDGE/COMMAND MERGE ==
  data: fuente input; py output size=[32 1]; py_python input; conectado input; py_estacion input; tg input
function py = fcn(fuente, py_python, conectado, py_estacion, tg)
%#codegen
% COMMAND MERGE: elige la fuente de comandos y completa los objetivos.
if fuente > 1.5
    % sin cliente queda el último paquete: el heartbeat deja de crecer
    % (-> PAUSED en MISSION), igual que con el puente real
    py = py_python + 0*conectado;
else
    py = py_estacion;
end
% Si la fuente no publica objetivos, los pone el detector simulado.
if py(4) < 0.5
    py(4) = tg(1);
    for i = 1:15
        py(4 + i) = tg(1 + i);
    end
end

== matlab function QD2_Sim_Dual/MISSION END (sim) ==
  data: estado input; parar output size=1; QD2_SIM parameter
function parar = fcn(estado, QD2_SIM)
%#codegen
% Detiene la simulación 3 s después de DONE (si QD2_SIM.parar_en_done = 1).
persistent n
if isempty(n), n = 0; end
if estado == 8
    n = n + 1;
else
    n = 0;
end
parar = double(QD2_SIM.parar_en_done > 0.5 && n >= 300);
